simulink model "si_wind_pdc"  (R2025b)
settings: Solver=FixedStepDiscrete  StartTime=0.0  StopTime=60  FixedStep=0.02  RelTol=1e-3
model workspace (MAT data in the model file):
  dt = 0.02
  initial_command = [4166666.66667; 0.0748583671255]
  initial_state = [0.278711869763; 4.60315878904; 0.00480231556131; 0; 0; 1.2; 1.2; 0.0748583671255]
  points(1).wind = 12
  points(1).state = [0.278711869763; 4.60315878904; 0.00480231556131; 0; 0; 1.2; 1.2; 0.0748583671255]
  points(1).command = [4166666.66667; 0.0748583671255]
  points(1).gain = [-786364.297801  -556024.569978  32390228.7398  294504.603792  67350.7556981  -29030670.0207  -67318886.4112  -271548.268038; 0.360195141728  -0.0455802356803  -6.39641194897  -0.313546151663  -0.040108202438  -1.27009308384  0.272924854828  0.967814107533]
  points(1).A = [0  0  0  1  0  0  0  0; 0  0  0  0  1  0  0  0; 0  0  0  0  0  0.999999999918  -0.999999999918  0; -4.53664175432  0.274684399071  0  -0.160232566141  0.13734219953  6.16557647458e-17  0  0; 4.53664175432  -9.29385012624  0  -5.2784732151  -10.0856308433  14.8073621666  0  -220.809035299; 0  0  -22.3853019567  -0.0239539838948  -0.0239539838876  -0.220719947424  0.160348915095  -0.403578425751; 0  0  172.652157155  0  0  1.23673051819  -1.23673051819  0; 0  0  0  0  0  0  0  -10]
  points(1).B = [0  0; 0  0; 0  0; 0  0; 0  0; 0  0; -1.98991233839e-07  0; 0  10]
  points(1).care_residual = 3.12444514705e-12
  points(1).max_pole_real = -0.395612627553
  points(2).wind = 14
  points(2).state = [0.215575570219; 3.56041018847; 0.00480231556131; 0; 0; 1.2; 1.2; 0.161044881395]
  points(2).command = [4166666.66667; 0.161044881395]
  points(2).gain = [-2083600.79795  -445149.868936  13833677.8002  530268.954192  78275.4776296  -20353406.8877  -65947067.557  -247830.29555; 0.203460398306  -0.0715429417961  -6.07188074796  -0.309981944435  -0.032211540351  -6.37991365492  0.24908664645  1.14783559628]
  points(2).A = [0  0  0  1  0  0  0  0; 0  0  0  0  1  0  0  0; 0  0  0  0  0  0.999999999918  -0.999999999918  0; -4.53664175432  0.274684399069  0  -0.160232566141  0.13734219953  -3.08278823729e-17  0  0; 4.53664175432  -9.2938501262  0  -5.10271838319  -9.90987600986  -7.88121180735  0  -251.668289335; 0  0  -22.3853019567  -0.0256249294026  -0.0256249293948  -0.280137618178  0.160348915095  -0.778303240496; 0  0  172.652157155  0  0  1.23673051819  -1.23673051819  0; 0  0  0  0  0  0  0  -10]
  points(2).B = [0  0; 0  0; 0  0; 0  0; 0  0; 0  0; -1.98991233839e-07  0; 0  10]
  points(2).care_residual = 2.94742008577e-12
  points(2).max_pole_real = -0.407302178838
  points(3).wind = 16
  points(3).state = [0.183925872349; 3.0376890534; 0.00480231556131; 0; 0; 1.2; 1.2; 0.22133752253]
  points(3).command = [4166666.66667; 0.22133752253]
  points(3).gain = [-2443868.80596  -372167.698717  -1456842.16803  645233.117588  74845.6207163  -13724634.2074  -64781367.6015  -333528.645718; 0.109768301806  -0.0765833448424  -7.75761275195  -0.293439165882  -0.0258210387603  -8.22988277058  0.335219435835  1.24544656582]
  points(3).A = [0  0  0  1  0  0  0  0; 0  0  0  0  1  0  0  0; 0  0  0  0  0  0.999999999918  -0.999999999918  0; -4.53664175432  0.274684399069  0  -0.160232566141  0.13734219953  0  0  -9.86492235933e-16; 4.53664175432  -9.2938501262  0  -5.31801451585  -10.125172146  -27.380926119  0  -264.443783501; 0  0  -22.3853019567  -0.0283607219264  -0.0283607219264  -0.359323067584  0.160348915095  -1.01982769205; 0  0  172.652157155  0  0  1.23673051819  -1.23673051819  0; 0  0  0  0  0  0  0  -10]
  points(3).B = [0  0; 0  0; 0  0; 0  0; 0  0; 0  0; -1.98991233839e-07  0; 0  10]
  points(3).care_residual = 2.00106597958e-12
  points(3).max_pole_real = -0.385324657835
  wind_data = [0 0.02 0.04 0.06 0.08 0.1 0.12 0.14 0.16 0.18 0.2 0.22 ... (6002 elements, 3001x2)]
settings Model: Creator=runner  LastModifiedBy=runner

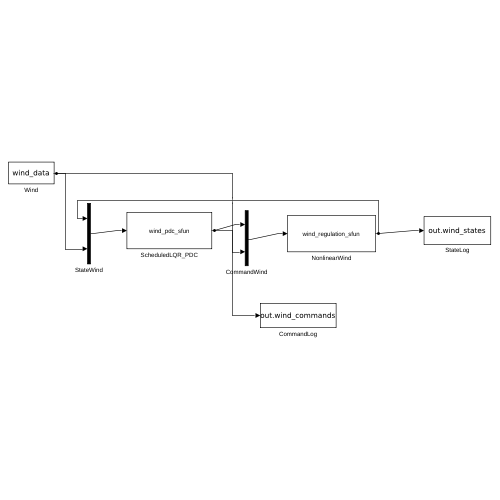
[thumbnail: Simulink's stored preview of the top-level diagram]
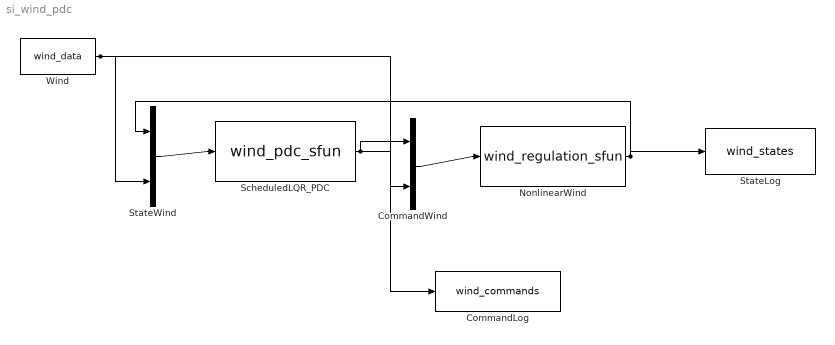
== system si_wind_pdc ==
  CommandLog : ToWorkspace  VariableName=wind_commands  SaveFormat=Structure With Time  SampleTime=-1
  CommandWind : Mux  Inputs=2
  NonlinearWind : S-Function  FunctionName=wind_regulation_sfun  Parameters=initial_state,dt  SFunctionDeploymentMode=off  EnableBusSupport=off
  ScheduledLQR_PDC : S-Function  FunctionName=wind_pdc_sfun  Parameters=points,initial_command,dt  SFunctionDeploymentMode=off  EnableBusSupport=off
  StateLog : ToWorkspace  VariableName=wind_states  SaveFormat=Structure With Time  SampleTime=-1
  StateWind : Mux  Inputs=2
  Wind : FromWorkspace  VariableName=wind_data  SampleTime=dt  Interpolate=off  OutputAfterFinalValue=Holding final value
  wires:
  Wind/1 -> StateWind/2, CommandWind/2
  NonlinearWind/1 -> StateWind/1, StateLog/1
  StateWind/1 -> ScheduledLQR_PDC/1
  ScheduledLQR_PDC/1 -> CommandWind/1, CommandLog/1
  CommandWind/1 -> NonlinearWind/1
